simulink model "stabilizer_bar_repair"  (R2023a)
settings: Solver=ode4  StartTime=0  StopTime=40  FixedStep=Ts_plant  MaxStep=0.001  RelTol=1e-3
InitFcn:
  | run(fullfile(fileparts(get_param(bdroot,'FileName')),'a001_new_Design_LQR_Controller.m'));
values from neighbouring files (symbols this model uses):
  cycle_cfg = jsondecode(fileread(fullfile(repair_root,'repair_support','repair_cycle_bank.json')))    [a001_new_Design_LQR_Controller.m]
  entry_cfg = rmfield(entry_bank_source,{'labels','source_hashes','note','source_par_sha256'})    [a001_new_Design_LQR_Controller.m]
  path_geometry = repair_build_geometry(path_cfg)    [a001_new_Design_LQR_Controller.m]
  path_Q = diag([10,10,2])    [a001_new_Design_LQR_Controller.m]
  path_R = diag([100,100,10])    [a001_new_Design_LQR_Controller.m]
  repair_cfg = struct    [a001_new_Design_LQR_Controller.m]
  repair_simfile = 'C:\Users\Public\Documents\CarSim2020.0_Data\Extensions\Simulink\00carsim_workspace\009\stabilizer_bar\simfile.sim'    [a001_new_Design_LQR_Controller.m]
  stadium_cfg = jsondecode(fileread(fullfile(repair_root,'repair_support','repair_stadium_reference.json')))    [a001_new_Design_LQR_Controller.m]
  Ts = 0.01    [a001_new_Design_LQR_Controller.m]
  Ts_plant = 0.0005    [a001_new_Design_LQR_Controller.m]
undefined symbols (not defined in the file or in its folder): path_cfg
(part 2 of 2)

== matlab function stabilizer_bar_repair/路径跟踪层/ContinuousProjection ==
  settings: updateMethod=DISCRETE  sampleTime=Ts
  data: X input; ey output size=1; Y input; psi input; beta input; alignment input size=[3 1]; DeltaChi output size=1; kappa output size=1; diag_project output size=[2 1]; path_geometry parameter; path_cfg parameter
function [ey,DeltaChi,kappa,diag_project] = path_projection(X,Y,psi,beta,alignment,path_geometry,path_cfg)
%#codegen
% 连续Frenet投影：只沿上一个弧长邻域迭代，弧长不取模存储，跨圈不跳点。
% ey为路径左侧正；DeltaChi为实际速度方向psi+beta与投影切向之差。
% 该投影用于式4.10；LQR仍跟踪时间索引参考，二者用途明确区分。
if path_cfg.feedback_enabled==0,ey=0;DeltaChi=0;kappa=0;diag_project=zeros(2,1);return;end
persistent s_prev
if isempty(s_prev),s_prev=0;end
c=cos(alignment(3));sn=sin(alignment(3));
dx=X-alignment(1);dy=Y-alignment(2);
x=c*dx+sn*dy;y=-sn*dx+c*dy;
s=s_prev;
% 牛顿投影的分母即1-kappa*ey；失效时停止，不夹紧分母。
for it=1:12
    [px,py,chi,k]=geometry(s,path_geometry,path_cfg);
    ex=x-px;ey0=y-py;
    lateral=-sin(chi)*ex+cos(chi)*ey0;
    den=1-k*lateral;
    % 分母状态只记录，不触发外加仿真停止。
    ds=(cos(chi)*ex+sin(chi)*ey0)/den;
    % 有界迭代步只用于局部求根，不能切换到全局另一段路径。
    s=s+ds;
    % 投影点跳变由路径误差和CarSim响应体现，不用Assert截断仿真。
    if abs(ds)<1e-7,break;end
end
[px,py,chi,kappa]=geometry(s,path_geometry,path_cfg);
ey=-sin(chi)*(x-px)+cos(chi)*(y-py);
tangential=cos(chi)*(x-px)+sin(chi)*(y-py);
% 切向投影残差保留在后续诊断中。
DeltaChi=atan2(sin(psi+beta-alignment(3)-chi),cos(psi+beta-alignment(3)-chi));
den=1-kappa*ey;
% 分母状态只记录，不触发外加仿真停止。
s_prev=s;diag_project=[s;den];
end
function [x,y,chi,k]=geometry(s,table,cfg)
if (cfg.mode==4 || cfg.mode==5),q=mod(s,cfg.length);else,q=s;end
[x,y,chi]=sample_geometry(q,table,cfg);
[k,~,~,~,~]=repair_path_profile(s,cfg);
end
function [x,y,chi]=sample_geometry(q,table,cfg)
% 均匀节点三次Hermite位置插值，切向由同一曲率积分生成。
ds=table(2,1)-table(1,1);j=min(max(floor(q/ds)+1,1),size(table,1)-1);
h=table(j+1,1)-table(j,1);u=(q-table(j,1))/h;
h00=2*u^3-3*u^2+1;h10=u^3-2*u^2+u;h01=-2*u^3+3*u^2;h11=u^3-u^2;
x=h00*table(j,2)+h10*h*cos(table(j,4))+h01*table(j+1,2)+h11*h*cos(table(j+1,4));
y=h00*table(j,3)+h10*h*sin(table(j,4))+h01*table(j+1,3)+h11*h*sin(table(j+1,4));
[~,~,~,~,chi]=repair_path_profile(q,cfg);
end

function [k,bw,dbds,stage,chi]=repair_path_profile(s,cfg)
% 曲率与侧偏角分别生成；chi是曲率对弧长的解析积分。
% mode=1入漂维持，2同步退出，3先恢复beta再退出，4原操场，5提前恢复beta操场。
L=cfg.transition;R=cfg.R;C=cfg.plateau;
% 普通轨迹：stage=1直线、2入弯、3恒曲率、4出弯、5末直线。
% 曲率与漂移权重独立；mode=6始终bw=0，不能只把beta设零。
if cfg.mode==6
 q=s-cfg.straight;bw=0;dbds=0;
 if q<=0,k=0;chi=0;stage=1;
 elseif q<L
  u=q/L;[h,~]=smooth(u);k=h/R;chi=L/R*primitive(u);stage=2;
 elseif q<L+C,k=1/R;chi=(q-L/2)/R;stage=3;
 elseif q<2*L+C
  u=(q-L-C)/L;[h,~]=smooth(u);k=(1-h)/R;chi=(L/2+C+L*(u-primitive(u)))/R;stage=4;
 else,k=0;chi=(L+C)/R;stage=5;end
 return;
end
if cfg.mode==4 || cfg.mode==5
 q=mod(s,cfg.half)-cfg.straight;half=floor(s/cfg.half);
 if q<=0,k=0;bw=0;dbds=0;stage=1;theta=0;
 elseif q<L
  u=q/L;[bw,db]=smooth(u);dbds=db/L;k=bw/R;stage=2;theta=L/R*primitive(u);
 elseif q<L+C
  k=1/R;bw=1;dbds=0;stage=3;theta=(q-L/2)/R;
  if cfg.mode==5 && q>L+C-L
   u=(q-(L+C-L))/L;[z,dz]=smooth(u);bw=1-z;dbds=-dz/L;stage=4;
  end
 else
  u=min((q-L-C)/L,1);[z,dz]=smooth(u);k=(1-z)/R;
  if cfg.mode==4,bw=1-z;dbds=-dz/L;else,bw=0;dbds=0;end
  stage=4;theta=(L/2+C+L*(u-primitive(u)))/R;
 end
 chi=pi*half+theta;stage=stage+4*mod(half,2);return;
end
% 入漂维持允许曲率与侧偏的建立长度/起点不同；chi仍只由曲率积分确定。
if cfg.mode==1
 q=s-cfg.straight;u=min(max(q/cfg.transition,0),1);[hk,~]=smooth(u);k=hk/cfg.R;
 if q<=0,chi=0;elseif q<cfg.transition,chi=cfg.transition/cfg.R*primitive(u);else,chi=(q-cfg.transition/2)/cfg.R;end
 v=min(max((q-cfg.beta_delay)/cfg.beta_transition,0),1);[bw,db]=smooth(v);dbds=db/cfg.beta_transition;
 if q<=0,stage=1;elseif u<1||v<1,stage=2;else,stage=3;end
 return;
end
q=s-cfg.straight;
if q<=0,k=0;bw=0;dbds=0;stage=1;chi=0;return;end
if q<L
 u=q/L;[bw,db]=smooth(u);dbds=db/L;k=bw/R;stage=2;chi=L/R*primitive(u);return;
end
k=1/R;bw=1;dbds=0;stage=3;chi=(q-L/2)/R;
if cfg.mode==1,return;end
% 独立退出站点由已通过3s稳态门槛的前置试验给出，不猜测稳定起点。
e=s-cfg.exit_s;if e<0,return;end
if cfg.mode==2
 u=min(e/L,1);[z,dz]=smooth(u);k=(1-z)/R;bw=1-z;dbds=-dz/L;
 chi=(cfg.exit_s-cfg.straight-L/2+L*(u-primitive(u)))/R;stage=4;
else
 u=min(e/L,1);[z,dz]=smooth(u);bw=1-z;dbds=-dz/L;stage=4;
 if e>=L
  z2=min((e-L)/L,1);[h,~]=smooth(z2);k=(1-h)/R;
  chi=(cfg.exit_s+L-cfg.straight-L/2+L*(z2-primitive(z2)))/R;stage=5;
 end
end
end
function [h,dh]=smooth(u)
h=10*u^3-15*u^4+6*u^5;dh=30*u^2*(1-u)^2;
end
function v=primitive(u)
v=2.5*u^4-3*u^5+u^6;
end

== matlab function stabilizer_bar_repair/CarSimInterface/FrontWheelActuator ==
  settings: updateMethod=DISCRETE  sampleTime=Ts_plant
  data: target input; left output; right output; left_rate output; right_rate output; diag output size=[6 1]; repair_cfg parameter
function [left,right,left_rate,right_rate,diag] = steer_direct(target,repair_cfg)
% 直接前轮输入，不叠加外部转角幅值或速率限制；角速度同步记录指令变化率。
persistent previous
if isempty(previous),previous=0;end
angle=target(1);
if repair_cfg.entry_mode==1,limit=repair_cfg.entry_steer_rate*repair_cfg.Ts_plant;angle=min(max(angle,previous-limit),previous+limit);end
rate=(angle-previous)/repair_cfg.Ts_plant;previous=angle;
left=angle*180/pi;right=left;left_rate=rate*180/pi;right_rate=left_rate;
diag=[angle;angle;angle;rate;0;0];
end

== matlab function stabilizer_bar_repair/CarSimInterface/InterfaceTestSelector ==
  settings: updateMethod=DISCRETE  sampleTime=Ts_plant
  data: command input size=[8 1]; u output size=[8 1]; t input; repair_interface_test parameter
function u=interface_selector(command,t,repair_interface_test)
% 仅在显式接口验证中产生2deg、10deg/s分段线性转角；其余时候透传。
u=command;
if repair_interface_test==0,return;end
knots=[0,.4,.6,.9,1.1,1.3,1.6,1.8,2,2.3,2.7,3,3.2,3.6];
left=[0,0,2,2,0,0,0,0,2,2,-2,-2,0,0];right=[0,0,0,0,0,-2,-2,0,2,2,-2,-2,0,0];
j=1;for k=1:13,if t>=knots(k),j=k;end;end
q=min(max((t-knots(j))/(knots(j+1)-knots(j)),0),1);
lr=(left(j+1)-left(j))/(knots(j+1)-knots(j));rr=(right(j+1)-right(j))/(knots(j+1)-knots(j));
u=[left(j)+q*(left(j+1)-left(j));right(j)+q*(right(j+1)-right(j));lr;rr;0;0;0;0];
end

== matlab function stabilizer_bar_repair/StageStop ==
  settings: updateMethod=DISCRETE  sampleTime=Ts
  data: valid input; stop output; plant input size=[50 1]; repair_interface_test parameter
function stop=stage_stop(valid,plant,repair_interface_test)
% 仅保留信号记录；候选、轮荷、查表告警不再触发自定义Stop Simulation。
stop=0;
end

== matlab function stabilizer_bar_repair/路径跟踪层/ReferenceAlignment ==
  settings: updateMethod=DISCRETE  sampleTime=Ts
  data: t input; ref output size=[14 1]; X input; Y input; psi input; V input; alignment output size=[3 1]; path_geometry parameter; path_cfg parameter
function [ref,alignment]=stadium_reference(t,X,Y,psi,V,path_geometry,path_cfg)
% 统一工况参考：初始实际质心对齐；入漂维持与两种退出独立选择。
% ref的14项接口与现有路径层保持一致，所有角度为rad。
persistent origin initial_speed
if isempty(origin),origin=[X;Y;psi];initial_speed=V;end
alignment=origin;T=path_cfg.ramp_time;u=min(max(t/T,0),1);H=10*u^3-15*u^4+6*u^5;
Vr=initial_speed+(path_cfg.V-initial_speed)*H;
if t<=T,s=initial_speed*t+(path_cfg.V-initial_speed)*T*(2.5*u^4-3*u^5+u^6);
else,s=(initial_speed+path_cfg.V)*T/2+path_cfg.V*(t-T);end
[k,bw,dbds,stage,chi]=repair_path_profile(s,path_cfg);
beta=path_cfg.beta*bw;bdot=path_cfg.beta*dbds*Vr;
if (path_cfg.mode==4 || path_cfg.mode==5),q=mod(s,path_cfg.length);lap=floor(s/path_cfg.length);else,q=s;lap=0;end
[x,y,~]=sample_geometry(q,path_geometry,path_cfg);
c=cos(origin(3));sn=sin(origin(3));chi=chi+origin(3);
ref=[origin(1)+c*x-sn*y;origin(2)+sn*x+c*y;chi-beta;Vr*cos(beta);Vr*sin(beta); ...
 k*Vr-bdot;Vr;beta;k;bw;stage;lap;s;chi];
end

function [x,y,chi]=sample_geometry(q,table,cfg)
% 均匀节点三次Hermite位置插值，切向由同一曲率积分生成。
ds=table(2,1)-table(1,1);j=min(max(floor(q/ds)+1,1),size(table,1)-1);
h=table(j+1,1)-table(j,1);u=(q-table(j,1))/h;
h00=2*u^3-3*u^2+1;h10=u^3-2*u^2+u;h01=-2*u^3+3*u^2;h11=u^3-u^2;
x=h00*table(j,2)+h10*h*cos(table(j,4))+h01*table(j+1,2)+h11*h*cos(table(j+1,4));
y=h00*table(j,3)+h10*h*sin(table(j,4))+h01*table(j+1,3)+h11*h*sin(table(j+1,4));
[~,~,~,~,chi]=repair_path_profile(q,cfg);
end

function [k,bw,dbds,stage,chi]=repair_path_profile(s,cfg)
% 曲率与侧偏角分别生成；chi是曲率对弧长的解析积分。
% mode=1入漂维持，2同步退出，3先恢复beta再退出，4原操场，5提前恢复beta操场。
L=cfg.transition;R=cfg.R;C=cfg.plateau;
% 普通轨迹：stage=1直线、2入弯、3恒曲率、4出弯、5末直线。
% 曲率与漂移权重独立；mode=6始终bw=0，不能只把beta设零。
if cfg.mode==6
 q=s-cfg.straight;bw=0;dbds=0;
 if q<=0,k=0;chi=0;stage=1;
 elseif q<L
  u=q/L;[h,~]=smooth(u);k=h/R;chi=L/R*primitive(u);stage=2;
 elseif q<L+C,k=1/R;chi=(q-L/2)/R;stage=3;
 elseif q<2*L+C
  u=(q-L-C)/L;[h,~]=smooth(u);k=(1-h)/R;chi=(L/2+C+L*(u-primitive(u)))/R;stage=4;
 else,k=0;chi=(L+C)/R;stage=5;end
 return;
end
if cfg.mode==4 || cfg.mode==5
 q=mod(s,cfg.half)-cfg.straight;half=floor(s/cfg.half);
 if q<=0,k=0;bw=0;dbds=0;stage=1;theta=0;
 elseif q<L
  u=q/L;[bw,db]=smooth(u);dbds=db/L;k=bw/R;stage=2;theta=L/R*primitive(u);
 elseif q<L+C
  k=1/R;bw=1;dbds=0;stage=3;theta=(q-L/2)/R;
  if cfg.mode==5 && q>L+C-L
   u=(q-(L+C-L))/L;[z,dz]=smooth(u);bw=1-z;dbds=-dz/L;stage=4;
  end
 else
  u=min((q-L-C)/L,1);[z,dz]=smooth(u);k=(1-z)/R;
  if cfg.mode==4,bw=1-z;dbds=-dz/L;else,bw=0;dbds=0;end
  stage=4;theta=(L/2+C+L*(u-primitive(u)))/R;
 end
 chi=pi*half+theta;stage=stage+4*mod(half,2);return;
end
% 入漂维持允许曲率与侧偏的建立长度/起点不同；chi仍只由曲率积分确定。
if cfg.mode==1
 q=s-cfg.straight;u=min(max(q/cfg.transition,0),1);[hk,~]=smooth(u);k=hk/cfg.R;
 if q<=0,chi=0;elseif q<cfg.transition,chi=cfg.transition/cfg.R*primitive(u);else,chi=(q-cfg.transition/2)/cfg.R;end
 v=min(max((q-cfg.beta_delay)/cfg.beta_transition,0),1);[bw,db]=smooth(v);dbds=db/cfg.beta_transition;
 if q<=0,stage=1;elseif u<1||v<1,stage=2;else,stage=3;end
 return;
end
q=s-cfg.straight;
if q<=0,k=0;bw=0;dbds=0;stage=1;chi=0;return;end
if q<L
 u=q/L;[bw,db]=smooth(u);dbds=db/L;k=bw/R;stage=2;chi=L/R*primitive(u);return;
end
k=1/R;bw=1;dbds=0;stage=3;chi=(q-L/2)/R;
if cfg.mode==1,return;end
% 独立退出站点由已通过3s稳态门槛的前置试验给出，不猜测稳定起点。
e=s-cfg.exit_s;if e<0,return;end
if cfg.mode==2
 u=min(e/L,1);[z,dz]=smooth(u);k=(1-z)/R;bw=1-z;dbds=-dz/L;
 chi=(cfg.exit_s-cfg.straight-L/2+L*(u-primitive(u)))/R;stage=4;
else
 u=min(e/L,1);[z,dz]=smooth(u);bw=1-z;dbds=-dz/L;stage=4;
 if e>=L
  z2=min((e-L)/L,1);[h,~]=smooth(z2);k=(1-h)/R;
  chi=(cfg.exit_s+L-cfg.straight-L/2+L*(z2-primitive(z2)))/R;stage=5;
 end
end
end
function [h,dh]=smooth(u)
h=10*u^3-15*u^4+6*u^5;dh=30*u^2*(1-u)^2;
end
function v=primitive(u)
v=2.5*u^4-3*u^5+u^6;
end

== matlab function stabilizer_bar_repair/EntryLocalMode/EntryLocalControl ==
  settings: updateMethod=DISCRETE  sampleTime=Ts
  data: y input size=[50 1]; command output size=[5 1]; t input; diag output size=[70 1]; entry_cfg parameter; repair_cfg parameter; cycle_diag output size=[16 1]; cycle_cfg parameter; stadium_packet input
function [command,diag,cycle_diag]=cycle_control(y,t,entry_cfg,repair_cfg,cycle_cfg,stadium_packet)
%#codegen
% 实际控制链：工作点/局部状态反馈→前轮角与轴滑移→公共轮速和转向执行。
% y为CarSim原50路采样输出，轮序FL/FR/RL/RR；command=[delta(rad);T四轮(Nm)]。
% entry_cfg冻结已验证起漂库；cycle_cfg含退出库、长度、维持时间和接管门槛。
% 原路径LQR与式4.10关闭。此函数不恢复车辆状态、不调用轮胎Fiala反演执行输入。
% diag保持原70项顺序；cycle_diag另记退出阶段、门控、进度与参考导数。
persistent phase distance elapsed readyTime captureTime satTime mix mixStart mixTarget mixElapsed prepareFailed vprev wprev initialized protection
persistent holdTime exitDistance straightCapture straightMix errors sats historyCount previousRef refInitialized
if isempty(initialized)
 phase=0;distance=0;elapsed=0;readyTime=0;captureTime=0;satTime=0;mix=0;mixStart=0;mixTarget=0;mixElapsed=0;prepareFailed=false;
 vprev=zeros(3,1);wprev=zeros(4,1);initialized=false;protection=false;
 holdTime=0;exitDistance=0;straightCapture=0;straightMix=0;errors=zeros(500,3);sats=false(500,1);historyCount=0;previousRef=zeros(7,1);refInitialized=false;
end
command=zeros(5,1);diag=zeros(70,1);cycle_diag=zeros(16,1);
if repair_cfg.entry_mode==0,return;end
Ts=repair_cfg.Ts;Rw=repair_cfg.Rw;Iw=repair_cfg.Iw;
x=[hypot(y(2),y(3))/3.6;y(4)*pi/180;y(5)*pi/180;mean(y(27:28));mean(y(29:30));y(8)*pi/180;y(26)*pi/180];
omega=y(21:24)*pi/30;Fz=y(17:20);last=entry_cfg.nodes(7);oldphase=phase;
assert(all(isfinite(x))&&all(isfinite(Fz)),'Nonfinite state or wheel load');first=~initialized;
if first,vprev=entry_cfg.normal.v;wprev=omega;initialized=true;end
elapsed=elapsed+Ts;if protection,satTime=satTime+Ts;else,satTime=0;end
errors(1:499,:)=errors(2:500,:);errors(500,:)=(x(1:3)-last.x(1:3))';sats(1:499)=sats(2:500);sats(500)=protection;historyCount=min(500,historyCount+1);
inside=all(abs(x-last.x)<=entry_cfg.thresholds)&&all(Fz>0)&&satTime<.2;
exitProgress=0;substage=0;holdgate=false;progress=smooth5(distance/entry_cfg.length);weight=0;ref=entry_cfg.normal;request=zeros(3,1);

% 操场模式由路径层提供唯一参考与反馈请求；共用下面唯一执行器历史。
if repair_cfg.stadium_mode==0
% 起漂段完全保留v0.1状态机和插值，新增退出仅在局部维持验收之后启用。
if phase<4
 if phase==0
  ready=abs(x(1)-12)<=.2&&abs(x(2))<=pi/180&&abs(x(3))<=.02;
  if ready,readyTime=readyTime+Ts;else,readyTime=0;end
  if readyTime>=1-1e-9&&~prepareFailed,phase=1;elseif elapsed>=10,prepareFailed=true;end
 else
  if phase==1,distance=distance+max(x(1),0)*Ts;end
  if inside,captureTime=captureTime+Ts;else,captureTime=0;end
  if phase==1&&captureTime>=.3-1e-9,phase=2;mixStart=mix;mixTarget=1;mixElapsed=0;end
  if (phase==2||phase==3)&&~inside&&mixTarget~=0,phase=2;mixStart=mix;mixTarget=0;mixElapsed=0;end
  if phase==2
   mixElapsed=mixElapsed+Ts;mix=mixStart+(mixTarget-mixStart)*smooth5(mixElapsed/.5);
   if mixElapsed>=.5-1e-9,if mixTarget==1,phase=3;else,phase=1;end,end
  end
 end
 progress=smooth5(distance/entry_cfg.length);
 if phase==0,ref=mixnode(entry_cfg.normal,entry_cfg.nodes(1),smooth5(t/2));
 else,ref=sampleNodes(entry_cfg.nodes,entry_cfg.grid,progress);end
 request=(1-mix)*(ref.v-feedback_delta(ref.K,x-ref.x))+mix*(last.v-feedback_delta(last.K,x-last.x));ref=mixnode(ref,last,mix);
 weight=mix;
 if phase==3&&oldphase==3,holdTime=holdTime+Ts;else,holdTime=0;end
 % drift_cycle保持末5秒门控；研究drift_turn按完整稳定弧验收，切换只检末0.5秒。
 historyRequired=500;if cycle_cfg.scheme==3,historyRequired=50;end
 if repair_cfg.cycle_mode==1&&holdTime>=cycle_cfg.hold_min_s-1e-8&&historyCount>=historyRequired
  tol=cycle_cfg.drift_tolerance;
  if cycle_cfg.scheme==3
   rmse=sqrt(mean(errors(451:500,:).^2,1))';trend=mean(errors(491:500,:),1)'-mean(errors(451:460,:),1)';
   satFraction=mean(double(sats(451:500)));firstHistory=451;
  else
   rmse=sqrt(mean(errors.^2,1))';trend=mean(errors(401:500,:),1)'-mean(errors(1:100,:),1)';
   satFraction=mean(double(sats));firstHistory=1;
  end
  run=0;longest=0;for k=firstHistory:500,if sats(k),run=run+1;else,run=0;end;longest=max(longest,run);end
  holdgate=all(rmse<=tol)&&all(abs(trend)<=tol)&&satFraction<=.05&&longest*Ts<=.2&&all(Fz>0);
  if holdgate,phase=4;exitDistance=0;end
 end
end

% 退出库独立。原B保持两段退出；scheme=3连接漂移点→r=.3普通弯→直行，滑移卸载与横摆下降重叠。
% 直行接管使用同一执行器历史，不复位车辆，也不叠加两套轮速环输出。
if phase>=4
 if phase==4&&oldphase>=4,exitDistance=exitDistance+max(x(1),0)*Ts;end
 q=min(exitDistance/cycle_cfg.length,1);
 if cycle_cfg.scheme==2
  if q<.5,exitProgress=.5*smooth5(2*q);else,exitProgress=.5+.5*smooth5(2*q-1);end
 else,exitProgress=smooth5(q);end
 if exitProgress<.5,substage=1;else,substage=2;end
 ref=sampleNodes(cycle_cfg.nodes,cycle_cfg.grid,exitProgress);normal=cycle_cfg.nodes(end);
 inside=all(abs(x-normal.x)<=cycle_cfg.straight_capture)&&all(Fz>0)&&~protection&&exitProgress>=1-1e-8;
 if inside,straightCapture=straightCapture+Ts;else,straightCapture=0;end
 if phase==4&&straightCapture>=.3-1e-8,phase=5;straightMix=0;end
 if phase==5
  straightMix=min(1,straightMix+Ts/.5);
  if ~inside,phase=4;elseif straightMix>=1-1e-8,phase=6;end
 end
 weight=0;if phase==5,weight=smooth5(straightMix);elseif phase==6,weight=1;end
 request=(1-weight)*(ref.v-feedback_delta(ref.K,x-ref.x))+weight*(normal.v-feedback_delta(normal.K,x-normal.x));ref=mixnode(ref,normal,weight);
end
else
 ref.x=stadium_packet(1:7);ref.v=stadium_packet(8:10);ref.offset=stadium_packet(11:14);ref.K=zeros(3,5);
 request=stadium_packet(15:17);phase=stadium_packet(18);progress=stadium_packet(19);mix=1;weight=1;
end
rates=zeros(7,1);if refInitialized,rates=(ref.x-previousRef)/Ts;end;previousRef=ref.x;refInitialized=true;
cycle_diag=[phase;exitProgress;substage;holdTime;double(holdgate);double(inside);straightCapture;weight;exitDistance;rates];

% 公共执行层：真实接地点速度、实际Fx负载补偿与冻结的局部执行预算。
lo=[ref.v(1)-entry_cfg.steer_deviation;entry_cfg.slip_low];hi=[ref.v(1)+entry_cfg.steer_deviation;entry_cfg.slip_high];
v=min(max(request,lo),hi);slew=[entry_cfg.steering_rate_rad_s;entry_cfg.slip_rate;entry_cfg.slip_rate];v=min(max(v,vprev-slew*Ts),vprev+slew*Ts);vprev=v;
contact=Rw*omega./(1+y(27:30));assert(all(isfinite(contact))&&all(contact>0),'Invalid contact velocity');
candidate=contact/Rw.*(1+[v(2);v(2);v(3);v(3)]);loadTorque=Rw*y(9:12)+ref.offset;kw=entry_cfg.wheel_kw;
if first,wd=omega;dwd=zeros(4,1);
else
 gain=kw+Iw/Ts;low=(-entry_cfg.torque_limit+kw*omega+Iw/Ts*wprev-loadTorque)/gain;high=(entry_cfg.torque_limit+kw*omega+Iw/Ts*wprev-loadTorque)/gain;
 low=max(low,wprev-entry_cfg.omega_acceleration*Ts);high=min(high,wprev+entry_cfg.omega_acceleration*Ts);assert(all(low<=high),'Empty torque and wheel acceleration budget');
 wd=min(max(candidate,low),high);dwd=(wd-wprev)/Ts;
end
feedback=kw*(wd-omega);inertia=Iw*dwd;raw=feedback+inertia+loadTorque;T=min(max(raw,-entry_cfg.torque_limit),entry_cfg.torque_limit);wprev=wd;
protection=any(abs(T)>=entry_cfg.torque_limit-1e-6);command=[v(1);T];
diag=[phase;progress;mix;double(inside);double(prepareFailed);readyTime;captureTime;satTime;x;ref.x;ref.v;request;v;candidate;wd;omega;feedback;inertia;loadTorque;raw;T;double(any(abs(v-request)>1e-9));double(any(abs(wd-candidate)>1e-9));double(protection);contact];
end
function h=smooth5(q)
q=min(max(q,0),1);h=10*q^3-15*q^4+6*q^5;
end
function out=mixnode(a,b,f)
out=a;out.x=(1-f)*a.x+f*b.x;out.v=(1-f)*a.v+f*b.v;out.K=(1-f)*a.K+f*b.K;out.offset=(1-f)*a.offset+f*b.offset;
end
function out=sampleNodes(nodes,grid,s)
j=1;for k=1:numel(grid)-1,if s>=grid(k),j=k;end,end
f=(s-grid(j))/(grid(j+1)-grid(j));out=mixnode(nodes(j),nodes(j+1),f);
end


function du=feedback_delta(K,error)
% 五项误差反馈：车辆侧倾仍存在，但不直接进入转角/滑移请求。
% K为3×5，状态前五项顺序为V、beta、AVz、前后轴滑移。
du=K*error(1:5);
end

== matlab function stabilizer_bar_repair/EntryModeSelector ==
  data: newcmd input size=[5 1]; angle output; oldcmd input size=[5 1]; tfl output; tfr output; trl output; trr output; repair_cfg parameter
function [angle,tfl,tfr,trl,trr]=select_commands(newcmd,oldcmd,repair_cfg)
% 模式开关只选择执行输入；不改变两支路的数学公式。
c=oldcmd;if repair_cfg.entry_mode==1,c=newcmd;end
angle=c(1);tfl=c(2);tfr=c(3);trl=c(4);trr=c(5);
end

== matlab function stabilizer_bar_repair/EntryLocalMode/EntryForceDiagnostic ==
  settings: updateMethod=DISCRETE  sampleTime=Ts
  data: y input size=[50 1]; out output size=[20 1]; diag input size=[70 1]; repair_cfg parameter
function out=entry_force_diagnostic(y,diag,repair_cfg)
%#codegen
% 本块仅记录原三自由度逆解回代及其与实际轮胎合力的差异，不参与执行指令。
% out=[原请求4;代数回代残差3;实际轴力4;实际平面合力矩3;请求平面合力矩3;差值3]。
% 实际合力矩使用四轮Fx/Fy、前轮实测角及轮距；未包含回正力矩/外倾/三维悬架作用。
persistent history initialized
if isempty(initialized),history=zeros(4,1);initialized=false;end
out=zeros(20,1);if repair_cfg.entry_mode==0,return;end
V=diag(9);beta=diag(10);r=diag(11);ref=diag(16:18);Ts=repair_cfg.Ts;
bd=ref(2);rd=ref(3);diffs=zeros(4,1);
if initialized,diffs=([bd;beta;rd;r]-history)/Ts;end
history=[bd;beta;rd;r];initialized=true;
vdot=repair_cfg.k_V*(ref(1)-V);betadot=repair_cfg.k_beta_p*(bd-beta)+repair_cfg.k_beta_d*(diffs(1)-diffs(2));
rdot=repair_cfg.k_r_p*(rd-r)+repair_cfg.k_r_d*(diffs(3)-diffs(4));q=betadot+r;
m=repair_cfg.m;Iz=repair_cfg.Iz;a=repair_cfg.a;b=repair_cfg.b;L=a+b;
angles=[y(38:39)*pi/180;0;0];delta=mean(angles(1:2));cd=cos(delta);sd=sin(delta);
Fxf=m*vdot;Fyr=(-Iz*rdot+a*m*V*q*cos(beta)+a*m*vdot*sin(beta))/L;
Fyf=(Iz*rdot-L*Fxf*sd+b*m*V*q*cos(beta)+b*m*vdot*sin(beta))/(L*cd);
Fxr=(-L*Fxf+Iz*rdot*sd-a*m*V*q*sin(beta)*cd-b*m*V*q*sin(beta-delta)+a*m*vdot*cos(beta)*cd+b*m*vdot*cos(beta-delta))/(L*cd);
bx=Fxf*cd-Fyf*sd+Fxr;by=Fxf*sd+Fyf*cd+Fyr;mz=a*(Fxf*sd+Fyf*cd)-b*Fyr;
back=[(bx*cos(beta)+by*sin(beta))/m;(-bx*sin(beta)+by*cos(beta))/(m*V)-r;mz/Iz];
Fx=y(9:12);Fy=y(13:16);cx=Fx.*cos(angles)-Fy.*sin(angles);cy=Fx.*sin(angles)+Fy.*cos(angles);
actual=[sum(cx);sum(cy);a*sum(cy(1:2))-b*sum(cy(3:4))+repair_cfg.d/2*(cx(2)-cx(1)+cx(4)-cx(3))];
request=[bx;by;mz];out=[Fxf;Fyf;Fxr;Fyr;back-[vdot;betadot;rdot];sum(Fx(1:2));sum(Fy(1:2));sum(Fx(3:4));sum(Fy(3:4));actual;request;actual-request];
end

== matlab function stabilizer_bar_repair/路径跟踪层/StadiumGuidance ==
  settings: updateMethod=DISCRETE  sampleTime=Ts
  data: y input; packet output; t input; stadium_diag output; stadium_cfg parameter; entry_cfg parameter; repair_cfg parameter; roll_feedback output; feedback_diag output
function [packet,stadium_diag,roll_feedback,feedback_diag]=stadium_guidance(y,t,stadium_cfg, entry_cfg, repair_cfg)
%#codegen
% 固定路线投影→阶段/局部工作点→小幅横摆修正；不直接驱动车轮。
% y：SI换算前CarSim50路；packet：参考状态7、前馈3、负载偏置4、请求3、阶段、进度。
% stadium_diag：s,bend,phase,ey,dChi,原始dr,限后dr,r_ref,r_modified,两限幅标志,
% 局部XY,chi_ref,gain,lap,切换失败。位置m，角度rad，角速度rad/s。
% 路线来源于已验收单弯，在试验前冻结；80m引入段不计入闭合路线。
persistent initialized previous chi j dr previousPhase failed failedPlanar failedRoll failedContact
feedback_diag=zeros(17,1);roll_feedback=zeros(6,1);packet=zeros(19,1);stadium_diag=zeros(17,1);
if repair_cfg.stadium_mode==0,return;end
c=stadium_cfg;h=c.angle;R=[cos(h),sin(h);-sin(h),cos(h)];
if isempty(initialized),previous=y(35:36);chi=(y(37)+y(4))*pi/180;j=1;dr=0;previousPhase=0;failed=false;failedPlanar=false;failedRoll=false;failedContact=false;initialized=true;end
point=R*(y(35:36)-c.origin);delta=y(35:36)-previous;
if norm(delta)>1e-8,chi=atan2(delta(2),delta(1));end;previous=y(35:36);
% 只在上一投影附近搜索，防止跳到对向直线。线段投影是有限区间内的最近点。
n=numel(c.s);low=max(1,j-20);high=min(n-1,j+39);best=inf;chosen=j;fraction=0;closest=zeros(2,1);
for k=low:high
 a=c.xy(k,:)';d=c.xy(k+1,:)'-a;f=min(max(dot(point-a,d)/dot(d,d),0),1);near=a+f*d;distance=sum((point-near).^2);
 if distance<best,best=distance;chosen=k;fraction=f;closest=near;end
end
j=chosen;f=fraction;s=(1-f)*c.s(j)+f*c.s(j+1);chiref=(1-f)*c.chi(j)+f*c.chi(j+1);
direction=R*[cos(chi);sin(chi)];localchi=atan2(direction(2),direction(1));dchi=atan2(sin(localchi-chiref),cos(localchi-chiref));
ey=dot(point-closest,[-sin(chiref);cos(chiref)]);
refx=((1-f)*c.x(j,:)+f*c.x(j+1,:))';refv=((1-f)*c.v(j,:)+f*c.v(j+1,:))';offset=((1-f)*c.offset(j,:)+f*c.offset(j+1,:))';
K=zeros(3,5);for a=1:3,for b=1:5,K(a,b)=(1-f)*c.K(j,a,b)+f*c.K(j+1,a,b);end,end
w=1; % 编译时显式定义初始混合权重，t>=2不混合。
if t<2
 q=min(max(t/2,0),1);w=10*q^3-15*q^4+6*q^5;
 refx=(1-w)*entry_cfg.normal.x+w*refx;refv=(1-w)*entry_cfg.normal.v+w*refv;offset=(1-w)*entry_cfg.normal.offset+w*offset;K=(1-w)*entry_cfg.normal.K+w*K;
end
% 行进方向反馈不是路径LQR。正ey/正方向误差时要求减少左转。
gain=c.g0+(c.g1-c.g0)*min(abs(refx(2))/(10*pi/180),1);
rawdr=-(c.wn^2/max(refx(1),1)*ey+2*c.wn*dchi)/gain;
target=min(max(rawdr,-c.correction_limit),c.correction_limit);dr=min(max(target,dr-c.correction_rate*repair_cfg.Ts),dr+c.correction_rate*repair_cfg.Ts);
x=[hypot(y(2),y(3))/3.6;y(4)*pi/180;y(5)*pi/180;mean(y(27:28));mean(y(29:30));y(8)*pi/180;y(26)*pi/180];
% 五项误差反馈与小幅横摆修正共用当前冻结K，不引入第二套执行命令。
% Roll/AVx仍记录并参与原接管门控；其连续反馈贡献固定为零。
request=refv-K*(x(1:5)-refx(1:5))+K(:,3)*dr;
roll_feedback=zeros(6,1); % 保留日志端口兼容，明确两项直接反馈均为零。
phase=c.phase(j);
% 位置到达但状态未就绪时记录任务失败，不推迟路线或重置车辆掩盖偏差。
if phase~=previousPhase
 if phase==3,failed=failed||any(abs(x-entry_cfg.nodes(end).x)>entry_cfg.thresholds)||any(y(17:20)<=0);end
 if phase==5,limit=[.2;pi/180;.02;.02;.04;2*pi/180;10*pi/180];failed=failed||any(abs(x-refx)>limit)||any(y(17:20)<=0);end
 % 原失败标志保留；新增分项使Roll偏差不会被误报为横纵向失效。
 if phase==3
  err=abs(x-entry_cfg.nodes(end).x);lim=entry_cfg.thresholds;
  failedPlanar=failedPlanar||any(err(1:5)>lim(1:5));
  failedRoll=failedRoll||any(err(6:7)>lim(6:7));
  failedContact=failedContact||any(y(17:20)<=0);
 elseif phase==5
  err=abs(x-refx);lim=[.2;pi/180;.02;.02;.04;2*pi/180;10*pi/180];
  failedPlanar=failedPlanar||any(err(1:5)>lim(1:5));
  failedRoll=failedRoll||any(err(6:7)>lim(6:7));
  failedContact=failedContact||any(y(17:20)<=0);
 end
end
% 前7项记录反馈维数与两项零贡献，随后为名义前馈、实际请求及失败分项。
feedback_diag=[5;zeros(6,1);refv;request;double(failedPlanar);double(failedRoll);double(failedContact);double(failed)];
previousPhase=phase;packet=[refx;refv;offset;request;phase;s/c.length];
stadium_diag=[s;c.bend(j);phase;ey;dchi;rawdr;dr;refx(3);refx(3)+dr;double(abs(rawdr)>c.correction_limit);double(abs(dr-target)>1e-9);point;chiref;gain;double(s>=c.length-1e-7);double(failed)];
end

== matlab function stabilizer_bar_repair/ActiveRollResearch/MomentDemand ==
  settings: updateMethod=DISCRETE  sampleTime=Ts_plant
  data: raw input; phi output; rate output; moment output; dk output; asb_cfg parameter
function [phi,rate,moment,dk]=asb_moment_demand(raw,asb_cfg)
%#codegen
% 理想主动稳定杆：只改变辅助侧倾恢复刚度，不改变主弹簧或漂移控制器。
% raw为CarSim新增26路输出；前2项相对侧倾deg，随后2项deg/s。
% moment为前后车体广义侧倾力矩Nm，正值增大对应相对侧倾；内部一律SI。
% 固定的是deltaK，不是力矩。软设置抵消部分内部384，硬设置增加恢复作用。
assert(all(isfinite(raw)),'ASB:Nonfinite suspension measurement');
phi=raw(1:2)*pi/180;rate=raw(3:4)*pi/180;
dk=asb_cfg.delta_K_deg*180/pi;
moment=-dk.*phi;
end

== matlab function stabilizer_bar_repair/ActiveRollResearch/ForcePair ==
  settings: updateMethod=DISCRETE  sampleTime=Ts_plant
  data: raw input; forces output; phi input; rate input; moment input; dk input; diag output; asb_cfg parameter
function [forces,diag]=asb_force_pair(raw,phi,rate,moment,dk,asb_cfg)
%#codegen
% 车体恢复力矩→等反轮端力→外部弹簧压缩力；轮序FL FR RL RR。
% raw(5:8)为FsExt[N]，9:12为Jnc[mm]，13:16为JncR[mm/s]，
% 17:20为CmpS[mm]，21:24为向内的SusY[mm]，25:26为内部Mx_A[Nm]。
% 正弹簧压缩力方向由独立正负100Nm短测核验；左正右负增大相对侧倾。
% 运动比dCmp/dJnc前0.959、后0.797。由虚功Fwheel=ratio*Fspring，
% 不能把轮端力直接写入IMP_FS。左右轮端等反，车体附加垂向合力为零。
lever=asb_cfg.track_m-[sum(raw(21:22));sum(raw(23:24))]*.001;
assert(all(lever>0)&&all(isfinite(moment)),'ASB:Invalid force-couple geometry');
q=moment./lever;wheel=[q(1);-q(1);q(2);-q(2)];forces=wheel./asb_cfg.motion_ratio;
% 读取CarSim实际收到的外部弹簧力，回代力偶与零合力；不用指令冒充实际量。
actual=raw(5:8);actualWheel=actual.*asb_cfg.motion_ratio;
actualMoment=[(actualWheel(1)-actualWheel(2))*lever(1)/2;(actualWheel(3)-actualWheel(4))*lever(2)/2];
net=[sum(actualWheel(1:2));sum(actualWheel(3:4))];
% 机械功两种口径独立记录：广义力矩×相对角速度，及弹簧力×压缩速度。
% 它们不等同电功率/耗电量；有限几何与交换采样误差通过差值暴露。
power=moment.*rate;jrate=raw(13:16)*.001;
powerSpring=-[sum(actualWheel(1:2).*jrate(1:2));sum(actualWheel(3:4).*jrate(3:4))];
geometricPhi=atan2([raw(10)-raw(9);raw(12)-raw(11)]*.001,lever);
% 44项诊断布局保存于信号说明；dM/dt来自固定刚度及实际角速度，首步无差分脉冲。
diag=[phi;rate;dk;moment;actualMoment;actualMoment-moment;lever;wheel;forces;actual;net;power;powerSpring;powerSpring-power;-dk.*rate;geometricPhi;geometricPhi-phi;raw(25:26);asb_cfg.target_K_deg];
end

== matlab function stabilizer_bar_repair/MATLAB Function ==
  settings: updateMethod=DISCRETE  sampleTime=Ts
  data: Vx input; V output; Vy input
function V = cg_speed(Vx,Vy)
%#codegen
V = hypot(Vx,Vy);
end

== matlab function stabilizer_bar_repair/路径跟踪层/PoseError ==
  settings: updateMethod=DISCRETE  sampleTime=Ts
  data: X input; xi output size=[3 1]; Y input; psi input; ref input size=[14 1]
function xi = pose_error(X,Y,psi,ref)
%#codegen
% 论文式4.4~4.8：全局位置误差为实际减参考，航向误差取主值。
% 参考psi保持连续累积，只有相对误差wrap，避免参考跨圈跳变。
xi=[X-ref(1);Y-ref(2);atan2(sin(psi-ref(3)),cos(psi-ref(3)))];
end

== matlab function stabilizer_bar_repair/路径跟踪层/OnlineLQR ==
  settings: updateMethod=DISCRETE  sampleTime=Ts
  data: ref input size=[14 1]; desired output size=[3 1]; xi input size=[3 1]; diag_lqr output size=[11 1]; path_Q parameter; path_R parameter; path_cfg parameter
function [desired,diag_lqr] = path_lqr(ref,xi,path_Q,path_R,path_cfg)
% 在线LQR目标直接输出；CARE残差保留诊断，不触发自定义Assert停止。
if path_cfg.feedback_enabled==0,desired=ref(4:6);diag_lqr=zeros(11,1);return;end
coder.extrinsic('lqr');c=cos(ref(3));s=sin(ref(3));vx=ref(4);vy=ref(5);
A=[0,0,-vx*s-vy*c;0,0,vx*c-vy*s;0,0,0];B=[c,-s,0;s,c,0;0,0,1];
K=zeros(3);P=zeros(3);[K,P]=lqr(A,B,path_Q,path_R);
AP=A'*P+P*A;PB=P*B*(path_R\(B'*P));
res=norm(AP-PB+path_Q,'fro')/(1+norm(AP,'fro')+norm(PB,'fro')+norm(path_Q,'fro'));
desired=ref(4:6)-K*xi;ok=all(isfinite(K(:)))&&isfinite(res)&&res<=path_cfg.care_tol;
diag_lqr=[K(:);res;double(ok)];
end

== matlab function stabilizer_bar_repair/车辆运动控制层/StateFeasibility ==
  settings: updateMethod=DISCRETE  sampleTime=Ts
  data: actual input size=[3 1]; packet output size=[13 1]; desired input size=[3 1]; delta input; loads input size=[2 1]; blend input; path input size=[3 1]; omega input size=[4 1]; contact input size=[8 1]; accepted output size=[3 1]; diag output size=[134 1]; valid output; repair_cfg parameter
function [packet,accepted,diag,valid] = state_governor(actual,desired,delta,loads,blend,path,omega,contact,repair_cfg)
% 直接把完整LQR状态参考送入原状态控制律，不做可行候选搜索或指令缩放。
% actual=[V;beta;r]，desired=[Vx_d;Vy_d;r_d]，path=[e_y;DeltaChi;kappa]；SI单位。
% 轮胎力可达性和执行器响应交由CarSim输出反映；diag只记录直通状态。
persistent history initialized
if isempty(initialized),history=zeros(4,1);initialized=false;end
V=actual(1);beta=actual(2);r=actual(3);
Vd=hypot(desired(1),desired(2));beta_d=atan2(desired(2),desired(1));r_d=desired(3);
eV=Vd-V;eBeta=atan2(sin(beta_d-beta),cos(beta_d-beta));eR=r_d-r;
if initialized
    beta_d_dot=atan2(sin(beta_d-history(1)),cos(beta_d-history(1)))/repair_cfg.Ts;
    beta_dot=atan2(sin(beta-history(2)),cos(beta-history(2)))/repair_cfg.Ts;
    r_d_dot=(r_d-history(3))/repair_cfg.Ts;r_dot=(r-history(4))/repair_cfg.Ts;
else
    beta_d_dot=0;beta_dot=0;r_d_dot=0;r_dot=0;
end
den=1-path(3)*path(1);
beta_cmd=repair_cfg.k_beta_p*eBeta+repair_cfg.k_beta_d*(beta_d_dot-beta_dot)+ ...
    repair_cfg.k_beta*path(3)*V*cos(path(2))/den;
r_cmd=repair_cfg.k_r_p*eR+repair_cfg.k_r_d*(r_d_dot-r_dot);
V_cmd=repair_cfg.k_V*eV;
packet=[Vd;beta_d;r_d;eV;eBeta;eR;beta_cmd;r_cmd;V_cmd;beta_d_dot;beta_dot;r_d_dot;r_dot];
accepted=desired;
valid=all(isfinite([actual;desired;delta;loads;blend;path;omega;contact;packet]));
diag=nan(134,1);diag(1)=1;diag(2)=double(valid);diag(3)=1;diag(4)=NaN;diag(5)=1;
diag(6:8)=desired;diag(9:11)=accepted;diag(100)=double(~valid);diag(101)=0;
history=[beta_d;beta;r_d;r];initialized=true;
end

== matlab function stabilizer_bar_repair/车辆运动控制层/RawDynamicsInverse ==
  settings: updateMethod=DISCRETE  sampleTime=Ts
  data: packet input size=[13 1]; F output size=[4 1]; delta input; Fzr input; blend input; actual input size=[3 1]; status output; repair_cfg parameter; residual output size=[3 1]
function [F,status,residual] = inverse_block(packet,delta,Fzr,blend,actual,repair_cfg)
% 三自由度动力学逆解输出未裁剪的轴级目标力，残差仅记录、不阻止执行。
qd=packet(7)+actual(3);V=actual(1);beta=actual(2);rdot=packet(8);Vdot=packet(9);
Fxf=repair_cfg.m*Vdot;cd=cos(delta);sd=sin(delta);L=repair_cfg.a+repair_cfg.b;
Fyr=(-repair_cfg.Iz*rdot+repair_cfg.a*repair_cfg.m*V*qd*cos(beta)+ ...
    repair_cfg.a*repair_cfg.m*Vdot*sin(beta))/L;
Fyf=(repair_cfg.Iz*rdot-L*Fxf*sd+repair_cfg.b*repair_cfg.m*V*qd*cos(beta)+ ...
    repair_cfg.b*repair_cfg.m*Vdot*sin(beta))/(L*cd);
Fxr=(-L*Fxf+repair_cfg.Iz*rdot*sd-repair_cfg.a*repair_cfg.m*V*qd*sin(beta)*cd- ...
    repair_cfg.b*repair_cfg.m*V*qd*sin(beta-delta)+repair_cfg.a*repair_cfg.m*Vdot*cos(beta)*cd+ ...
    repair_cfg.b*repair_cfg.m*Vdot*cos(beta-delta))/(L*cd);
F=[Fxf;Fyf;Fxr;Fyr];bx=F(1)*cd-F(2)*sd+F(3);by=F(1)*sd+F(2)*cd+F(4);
Vdot_back=(bx*cos(beta)+by*sin(beta))/repair_cfg.m;
beta_dot_back=(-bx*sin(beta)+by*cos(beta))/(repair_cfg.m*V)-actual(3);
r_dot_back=(repair_cfg.a*(F(1)*sd+F(2)*cd)-repair_cfg.b*F(4))/repair_cfg.Iz;
residual=[Vdot_back-packet(9);beta_dot_back-packet(7);r_dot_back-packet(8)];
status=int8(0); %#ok<NASGU> 保留原状态端口，力能否实现以CarSim实际响应判断。
end

== matlab function stabilizer_bar_repair/车辆运动控制层/ForceCorrection ==
  settings: updateMethod=DISCRETE  sampleTime=Ts
  data: F input size=[4 1]; alpha output; actual input size=[3 1]; delta input; loads input size=[2 1]; wf output; wr output; Fxf output; Fxr output; diag output size=[32 1]; valid output; repair_cfg parameter
function [alpha,wf,wr,Fxf,Fxr,diag,valid] = force_block(F,actual,delta,loads,repair_cfg)
% 轴力不做摩擦圆、被动方向或前轮可达角投影；CarSim轮胎力是实际响应。
% alpha采用未饱和小侧偏斜率反算，只生成前轮指令；原始Fx用于轮速/力矩前馈。
% 轮速逆解使用载荷尺度的连续正则化，避免Fy过零时突变；它不是轮胎力/力矩限幅。
V=actual(1);beta=actual(2);r=actual(3);vx=V*cos(beta);vy=V*sin(beta);
contact=atan2(vy+repair_cfg.a*r,vx);alpha=-F(2)/repair_cfg.Caf;
vxf=vx*cos(delta)+(vy+repair_cfg.a*r)*sin(delta);
vyf=-vx*sin(delta)+(vy+repair_cfg.a*r)*cos(delta);vyr=vy-repair_cfg.b*r;
ef=repair_cfg.force_eps_frac*repair_cfg.mu*loads(1);
er=repair_cfg.force_eps_frac*repair_cfg.mu*loads(2);
wf=(vxf-vyf*F(1)*F(2)/(F(2)^2+ef^2))/repair_cfg.Rw;
wr=(vx-vyr*F(3)*F(4)/(F(4)^2+er^2))/repair_cfg.Rw;
Fxf=F(1);Fxr=F(3);valid=all(isfinite([F;actual;delta;loads;alpha;wf;wr]));
body=zeros(3,1);diag=[F;F;zeros(4,1);body;contact-alpha;contact-alpha;ef;er; ...
    ef^2/(F(2)^2+ef^2);er^2/(F(4)^2+er^2);0;0;vxf;vyf;vx;vyr;F(4)*vyr; ...
    repair_cfg.mu*loads(1);repair_cfg.mu*loads(2);NaN;double(~valid)];
end
